simulink library "Contact_Forces_Lib"  (R2024a)
settings: Solver=ode45  StartTime=0.0  StopTime=10.0  RelTol=1e-3  EnableMultiTasking=on
undefined symbols (not defined in the file or in its folder): b_contact, custom_param_1, custom_param_2, Extr_Data_Ring, k_contact, l_cone, length_cylinder, length_tube, mu_kinetic, mu_static, pen_exponent, pen_full_damp_F, rad_s_cone, radius_cylinder, radius_tube, v_thr, X, Y, Z
libraries: nesl_utility x197, sm_lib x115, $bdroot x72, simulink x20, fl_lib x4
(part 4 of 12)

== system Contact_Forces_Lib/3D/Composite Forces ==
  Face to Belt Faces Force : Subsystem  mask(Face to Belt Faces Force){PlaB_x=4, PlaB_y=1, PlaB_z=0.1, FacF_x=0.6, FacF_y=0.6, FacF_z=-0.6/2, FacF_rSph=0.03, force_law_pla2pla=Linear, k_contact_pla2pla=1e4, b_contact_pla2pla=1e2, pen_full_damp_F_pla2pla=1e-4, pen_exponent_pla2pla=1, friction_law_pla2pla=Stick-Slip Continuous, mu_kinetic_pla2pla=0.5, mu_static_pla2pla=0.7, v_thr_pla2pla=0.001, vis_on_pla2pla=off, vis_opc_en_box2box=0, vis_len_plaLz=0.0005, vis_clr=[0.9 0.2 0.2], vis_opc=0.7}
      mask prompts: PlaB_x "PlaB Length x (m)"; PlaB_y "PlaB Length y (m)"; PlaB_z "PlaB Depth to Reference Frame (m)"; FacF_x "FacF Length x (m)"; FacF_y "FacF Length y (m)"; FacF_z "FacF Depth to Reference Frame (m) (+/-)"; FacF_rSph "FacF Sphere Radius"; force_law_pla2pla "Force Law"; k_contact_pla2pla "Contact Stiffness (N/m)"; b_contact_pla2pla "Contact Damping (N/(m/s))"; pen_full_damp_F_pla2pla "Penetration for full damping (m)"; pen_exponent_pla2pla "Penetration exponent (>=1)"; friction_law_pla2pla "Friction Law"; mu_kinetic_pla2pla "Coefficient of Kinetic Friction"; mu_static_pla2pla "Coefficient of Static Friction"; v_thr_pla2pla "Velocity Threshold (m/s)"; vis_on_pla2pla "Visualize Contact Surfaces"; vis_opc_en_box2box "Visualize Opacity Enable"; vis_len_plaLz "Depth Plane Surface Element (Z-Axis) (m)"; vis_clr "Color of Surface Element (RGB)"; vis_opc "Opacity of Surface Element (0-1)"
      mask help:
      | This subsystem models planar contact forces between a square face and a conveyor belt.  The conveyor belt moves at the speed specified by the input signal in m/s.  Velocity can be specified along x or y and affects upper and lower surfaces of the belt.
      |
      | Frame connected to PlaB port:
      | 1. Located at midpoint of plane (x, y, and z).
      | 2. Z-axis is normal to the surfaces where force is active.
      |
      | Frame connected to the FacF port:
      | 1. Located at midpoint of box (x, y, and z).
      | 2. Z-axis is normal to the surfaces where force is active.
      |
      | Output signal is a bus with intermediate calculations and total force.
      mask init:
      | f=Simulink.FindOptions('FollowLinks',0,'LookUnderMasks','none','RegExp',1);
      | CR_bpth=Simulink.findBlocks(gcb,'friction_law','.*',f);
      | if(~isempty(CR_bpth))
      |     temp_frlaw = get_param(gcb,'friction_law_pla2pla');
      |     for i=1:length(CR_bpth)
      |         set_param(CR_bpth(i),'friction_law',temp_frlaw);
      |     end
      |     clear temp_frlaw
      | 
      |     temp_forcelaw = get_param(gcb,'force_law_pla2pla');
      |     for i=1:length(CR_bpth)
      |         set_param(CR_bpth(i),'force_law',temp_forcelaw);
      |     end
      |     clear temp_forcelaw
      | 
      |     temp_vis_on = get_param(gcb,'vis_on_pla2pla');
      |     for i=1:length(CR_bpth)
      |         set_param(CR_bpth(i),'vis_on',temp_vis_on);
      |     end
      |     clear temp_vis_on
      | end
      mask Help: web(which('Face_to_Plane_Contact.html'));
      mask TypeOptions force_law_pla2pla: Linear | Nonlinear
      mask Callback force_law_pla2pla:
      | maskObj = Simulink.Mask.get(gcb);
      | pfd_h = maskObj.getParameter('pen_full_damp_F_pla2pla');
      | pex_h = maskObj.getParameter('pen_exponent_pla2pla');
      | if strcmp(get_param(gcb,'force_law_pla2pla'),'Linear')
      |     pfd_h.Visible = 'off';
      |     pex_h.Visible = 'off';
      | elseif strcmp(get_param(gcb,'force_law_pla2pla'),'Nonlinear')
      |     pfd_h.Visible = 'on';
      |     pex_h.Visible = 'on';
      | end
      mask TypeOptions friction_law_pla2pla: None | Stick-Slip Continuous
      mask Callback friction_law_pla2pla:
      | maskObj = Simulink.Mask.get(gcb);
      | muk_h = maskObj.getParameter('mu_kinetic_pla2pla');
      | mus_h = maskObj.getParameter('mu_static_pla2pla');
      | vth_h = maskObj.getParameter('v_thr_pla2pla');
      | if strcmp(get_param(gcb,'friction_law_pla2pla'),'None')
      |     muk_h.Visible = 'off';
      |     mus_h.Visible = 'off';
      |     vth_h.Visible = 'off';
      | elseif strcmp(get_param(gcb,'friction_law_pla2pla'),'Stick-Slip Continuous')
      |     muk_h.Visible = 'on';
      |     mus_h.Visible = 'on';
      |     vth_h.Visible = 'on';
      | end
      | clear maskObj
      mask Callback vis_on_pla2pla:
      | maskObj = Simulink.Mask.get(gcb);
      | vis_clr_h = maskObj.getParameter('vis_clr');
      | vis_opc_h = maskObj.getParameter('vis_opc');
      | vis_len_plaLz_h = maskObj.getParameter('vis_len_plaLz');
      | if strcmp(get_param(gcb,'vis_on_pla2pla'),'off')
      |     vis_len_plaLz_h.Visible = 'off';
      |     vis_clr_h.Visible = 'off';
      |     vis_opc_h.Visible = 'off';
      | elseif strcmp(get_param(gcb,'vis_on_pla2pla'),'on')
      |     vis_len_plaLz_h.Visible = 'on';
      |     vis_clr_h.Visible = 'on';
      |     vis_opc_h.Visible = 'on';
      | end
      | clear maskObj vis_clr_h vis_opc_h
      | clear vis_len_plaLz_h
      mask DialogControl Container6 Prompt: Dimensions
      mask DialogControl Container7 Prompt: Contact
      mask DialogControl Container9 Prompt: Friction
      mask DialogControl Vis_Cont Prompt: Visual
      mask Display: image('Face_to_Belt_Faces_IMAGE.jpg');
  Face to Plane Force : Subsystem  mask(Face to Plane Force){PlaB_x=1, PlaB_y=1, PlaB_z=0.05, FacF_x=0.1, FacF_y=0.1, FacF_z=0.05, FacF_rSph=0.01, force_law_pla2pla=Linear, k_contact_pla2pla=1e4, b_contact_pla2pla=1e2, pen_full_damp_F_pla2pla=1e-4, pen_exponent_pla2pla=1, friction_law_pla2pla=None, mu_kinetic_pla2pla=0.5, mu_static_pla2pla=0.7, v_thr_pla2pla=0.001, vis_on_pla2pla=off, vis_opc_en_box2box=0, vis_len_plaLz=0.005, vis_clr=[0.9 0.2 0.2], vis_opc=0.7}
      mask prompts: PlaB_x "PlaB Length x (m)"; PlaB_y "PlaB Length y (m)"; PlaB_z "PlaB Depth to Reference Frame (m)"; FacF_x "FacF Length x (m)"; FacF_y "FacF Length y (m)"; FacF_z "FacF Depth to Reference Frame (m) (+/-)"; FacF_rSph "FacF Sphere Radius"; force_law_pla2pla "Force Law"; k_contact_pla2pla "Contact Stiffness (N/m)"; b_contact_pla2pla "Contact Damping (N/(m/s))"; pen_full_damp_F_pla2pla "Penetration for full damping (m)"; pen_exponent_pla2pla "Penetration exponent (>=1)"; friction_law_pla2pla "Friction Law"; mu_kinetic_pla2pla "Coefficient of Kinetic Friction"; mu_static_pla2pla "Coefficient of Static Friction"; v_thr_pla2pla "Velocity Threshold (m/s)"; vis_on_pla2pla "Visualize Contact Surfaces"; vis_opc_en_box2box "Visualize Opacity Enable"; vis_len_plaLz "Depth Plane Surface Element (Z-Axis) (m)"; vis_clr "Color of Surface Element (RGB)"; vis_opc "Opacity of Surface Element (0-1)"
      mask help:
      | This subsystem implements a contact force between a plane and a square face. The plane is assumed significantly larger than the face such that the edges will never intersect.  The force is active above and below the plane and face.
      |
      | Frame connected to PlaB port:
      | 1. Located at midpoint of plane (x, y, and z).
      | 2. Z-axis is normal to the surfaces where force is active.
      |
      | Frame connected to the FacF port:
      | 1. Located at midpoint of box (x, y, and z).
      | 2. Z-axis is normal to the surfaces where force is active.
      |
      | Output signal is a bus with intermediate calculations and total force.
      mask init:
      | f=Simulink.FindOptions('FollowLinks',0,'LookUnderMasks','none','RegExp',1);
      | CR_bpth=Simulink.findBlocks(gcb,'friction_law','.*',f);
      | 
      | if(~isempty(CR_bpth))
      |     temp_frlaw = get_param(gcb,'friction_law_pla2pla');
      |     for i=1:length(CR_bpth)
      |         set_param(CR_bpth(i),'friction_law',temp_frlaw);
      |     end
      |     clear temp_frlaw
      | 
      |     temp_forcelaw = get_param(gcb,'force_law_pla2pla');
      |     for i=1:length(CR_bpth)
      |         set_param(CR_bpth(i),'force_law',temp_forcelaw);
      |     end
      |     clear temp_forcelaw
      | 
      |     temp_vis_on = get_param(gcb,'vis_on_pla2pla');
      |     for i=1:length(CR_bpth)
      |         set_param(CR_bpth(i),'vis_on',temp_vis_on);
      |     end
      |     clear temp_vis_on
      | end
      mask Help: web(which('Face_to_Plane_Contact.html'));
      mask TypeOptions force_law_pla2pla: Linear | Nonlinear
      mask Callback force_law_pla2pla:
      | maskObj = Simulink.Mask.get(gcb);
      | pfd_h = maskObj.getParameter('pen_full_damp_F_pla2pla');
      | pex_h = maskObj.getParameter('pen_exponent_pla2pla');
      | if strcmp(get_param(gcb,'force_law_pla2pla'),'Linear')
      |     pfd_h.Visible = 'off';
      |     pex_h.Visible = 'off';
      | elseif strcmp(get_param(gcb,'force_law_pla2pla'),'Nonlinear')
      |     pfd_h.Visible = 'on';
      |     pex_h.Visible = 'on';
      | end
      mask TypeOptions friction_law_pla2pla: None | Stick-Slip Continuous
      mask Callback friction_law_pla2pla:
      | maskObj = Simulink.Mask.get(gcb);
      | muk_h = maskObj.getParameter('mu_kinetic_pla2pla');
      | mus_h = maskObj.getParameter('mu_static_pla2pla');
      | vth_h = maskObj.getParameter('v_thr_pla2pla');
      | if strcmp(get_param(gcb,'friction_law_pla2pla'),'None')
      |     muk_h.Visible = 'off';
      |     mus_h.Visible = 'off';
      |     vth_h.Visible = 'off';
      | elseif strcmp(get_param(gcb,'friction_law_pla2pla'),'Stick-Slip Continuous')
      |     muk_h.Visible = 'on';
      |     mus_h.Visible = 'on';
      |     vth_h.Visible = 'on';
      | end
      | clear maskObj
      mask Callback vis_on_pla2pla:
      | maskObj = Simulink.Mask.get(gcb);
      | vis_clr_h = maskObj.getParameter('vis_clr');
      | vis_opc_h = maskObj.getParameter('vis_opc');
      | vis_len_plaLz_h = maskObj.getParameter('vis_len_plaLz');
      | if strcmp(get_param(gcb,'vis_on_pla2pla'),'off')
      |     vis_len_plaLz_h.Visible = 'off';
      |     vis_clr_h.Visible = 'off';
      |     vis_opc_h.Visible = 'off';
      | elseif strcmp(get_param(gcb,'vis_on_pla2pla'),'on')
      |     vis_len_plaLz_h.Visible = 'on';
      |     vis_clr_h.Visible = 'on';
      |     vis_opc_h.Visible = 'on';
      | end
      | clear maskObj vis_clr_h vis_opc_h
      | clear vis_len_plaLz_h
      mask DialogControl Container6 Prompt: Dimensions
      mask DialogControl Container7 Prompt: Contact
      mask DialogControl Container9 Prompt: Friction
      mask DialogControl Vis_Cont Prompt: Visual
      mask Display: image('Face_to_Plane_Contact_IMAGE.jpg');
  Sphere to Belt Force : Subsystem  mask(Sphere to Belt Force){sph_rad=1.6, belt_h=1, belt_w=3, belt_l=10, force_law_sph2bel=Linear, k_contact_sph2bel=5e5, b_contact_sph2bel=1e6, pen_full_damp_F_sph2bel=1*1e-2, pen_exponent_sph2bel=1, friction_law_sph2bel=Stick-Slip Continuous, mu_kinetic_sph2bel=0.5, mu_static_sph2bel=0.7, v_thr_sph2bel=1e-3, vis_on_sph2bel=off, vis_opc_en_sph2bel=0, vis_depth_sph2bel=1*0.01, vis_clr=[0.9 0.2 0.2], vis_opc=0.7}
      mask prompts: sph_rad "Sphere Radius (m)"; belt_h "Belt Height (m)"; belt_w "Belt Width (m)"; belt_l "Belt Length (m)"; force_law_sph2bel "Force Law"; k_contact_sph2bel "Contact Stiffness (N/m)"; b_contact_sph2bel "Contact Damping (N/(m/s))"; pen_full_damp_F_sph2bel "Penetration for full damping (m)"; pen_exponent_sph2bel "Penetration exponent (>=1)"; friction_law_sph2bel "Friction Law"; mu_kinetic_sph2bel "Coefficient of Kinetic Friction"; mu_static_sph2bel "Coefficient of Static Friction"; v_thr_sph2bel "Velocity Threshold (m/s)"; vis_on_sph2bel "Visualize Contact Surfaces"; vis_opc_en_sph2bel "Visualize Opacity Enable"; vis_depth_sph2bel "Depth Surface Element (m)"; vis_clr "Color of Surface Element (RGB)"; vis_opc "Opacity of Surface Element (0-1)"
      mask help:
      | This subsystem models contact forces between a sphere and a conveyor belt.  The conveyor belt moves at the speed specified by the input signal in m/s.  The speed and affects upper and lower surfaces of the belt as well as the ends.
      |
      | Frame connected to BelB port:
      | 1. Located at midpoint of plane (x, y, and z).
      | 2. Z-axis is normal to the surfaces where force is active.
      |
      | Frame connected to the SphF port:
      | 1. Located at center of sphere.
      | 2. Orientation does not matter.
      |
      | Output signal is a bus with intermediate calculations and total force. Click Help for a diagram describing this force.
      mask init:
      | f=Simulink.FindOptions('FollowLinks',0,'LookUnderMasks','none','RegExp',1);
      | CR_bpth=Simulink.findBlocks(gcb,'friction_law','.*',f);
      | 
      | if(~isempty(CR_bpth))
      |     temp_frlaw = get_param(gcb,'friction_law_sph2bel');
      |     for i=1:length(CR_bpth)
      |         set_param(CR_bpth(i),'friction_law',temp_frlaw);
      |     end
      |     clear temp_frlaw
      | 
      |     temp_forcelaw = get_param(gcb,'force_law_sph2bel');
      |     for i=1:length(CR_bpth)
      |         set_param(CR_bpth(i),'force_law',temp_forcelaw);
      |     end
      |     clear temp_forcelaw
      | 
      |     temp_vis_on = get_param(gcb,'vis_on_sph2bel');
      |     for i=1:length(CR_bpth)
      |         set_param(CR_bpth(i),'vis_on',temp_vis_on);
      |     end
      |     clear temp_vis_on
      | end
      mask Help: web(which('Sphere_to_Belt_Contact.html'));
      mask TypeOptions force_law_sph2bel: Linear | Nonlinear
      mask Callback force_law_sph2bel:
      | maskObj = Simulink.Mask.get(gcb);
      | pfd_h = maskObj.getParameter('pen_full_damp_F_sph2bel');
      | pex_h = maskObj.getParameter('pen_exponent_sph2bel');
      | if strcmp(get_param(gcb,'force_law_sph2bel'),'Linear')
      |     pfd_h.Visible = 'off';
      |     pex_h.Visible = 'off';
      | elseif strcmp(get_param(gcb,'force_law_sph2bel'),'Nonlinear')
      |     pfd_h.Visible = 'on';
      |     pex_h.Visible = 'on';
      | end
      mask Callback pen_full_damp_F_sph2bel:
      | maskObj = Simulink.Mask.get(gcb);
      | pfd_h = maskObj.getParameter('pen_full_damp_F_sph2bel');
      | pex_h = maskObj.getParameter('pen_exponent_sph2bel');
      | if strcmp(get_param(gcb,'force_law_sph2bel'),'Linear')
      |     pfd_h.Visible = 'off';
      |     pex_h.Visible = 'off';
      | elseif strcmp(get_param(gcb,'force_law_sph2bel'),'Nonlinear')
      |     pfd_h.Visible = 'on';
      |     pex_h.Visible = 'on';
      | end
      mask TypeOptions friction_law_sph2bel: None | Stick-Slip Continuous
      mask Callback friction_law_sph2bel:
      | maskObj = Simulink.Mask.get(gcb);
      | muk_h = maskObj.getParameter('mu_kinetic_sph2bel');
      | mus_h = maskObj.getParameter('mu_static_sph2bel');
      | vth_h = maskObj.getParameter('v_thr_sph2bel');
      | if strcmp(get_param(gcb,'friction_law_sph2bel'),'None')
      |     muk_h.Visible = 'off';
      |     mus_h.Visible = 'off';
      |     vth_h.Visible = 'off';
      | elseif strcmp(get_param(gcb,'friction_law_sph2bel'),'Stick-Slip Continuous')
      |     muk_h.Visible = 'on';
      |     mus_h.Visible = 'on';
      |     vth_h.Visible = 'on';
      | end
      | clear maskObj
      mask Callback vis_on_sph2bel:
      | maskObj = Simulink.Mask.get(gcb);
      | vis_clr_h = maskObj.getParameter('vis_clr');
      | vis_opc_h = maskObj.getParameter('vis_opc');
      | vis_depth_sph2bel_h = maskObj.getParameter('vis_depth_sph2bel');
      | if strcmp(get_param(gcb,'vis_on_sph2bel'),'off')
      |     vis_depth_sph2bel_h.Visible = 'off';
      |     vis_clr_h.Visible = 'off';
      |     vis_opc_h.Visible = 'off';
      | elseif strcmp(get_param(gcb,'vis_on_sph2bel'),'on')
      |     vis_depth_sph2bel_h.Visible = 'on';
      |     vis_clr_h.Visible = 'on';
      |     vis_opc_h.Visible = 'on';
      | end
      | clear maskObj vis_clr_h vis_opc_h
      | clear vis_depth_sph2bel_h
      mask DialogControl cont_dimensions Prompt: Dimensions
      mask DialogControl cont_contact Prompt: Contact
      mask DialogControl cont_friction Prompt: Friction
      mask DialogControl cont_vis Prompt: Visual
      mask Display: image('Sphere_to_Belt_IMAGE.jpg');

== system Contact_Forces_Lib/3D/Prototype ==
  note: These blocks are prototypes, and will change in future releases.
      | They are provided as an example.
  Cone in Ring Force : Subsystem  mask{r_cyl=radius_cylinder, l_cyl=length_cylinder, r_tube=radius_tube, l_tube=length_tube, rl=radius_cylinder, rs=rad_s_cone, lc=l_cone, k_stiff=k_contact, b_damp=b_contact, n=500}
      mask prompts: r_cyl "Cylinder radius (m)"; l_cyl "Cylinder length"; r_tube "Tube radius (m)"; l_tube "Tube length (m)"; rl "Cone Large radius (m)"; rs "Cone Small radius (m)"; lc "Cone Length"; k_stiff "Spring Stifness (N/m)"; b_damp "Damping (Ns/m)"; n "Number of discrete points"
      mask DialogControl Dim Prompt: Dimensions
      mask DialogControl contact Prompt: Contact Forces
      mask Display:
      | port_label('LConn',1,'TubB');
      | port_label('RConn',1,'CylF');
  Cylinder In Ring Force : Subsystem  mask{r_cyl=radius_cylinder, l_cyl=length_cylinder, r_tube=radius_tube, l_tube=length_tube, k_stiff=k_contact, b_damp=b_contact, n=500, mu_kinetic=mu_kinetic, mu_static=mu_static, v_thr=v_thr}
      mask prompts: r_cyl "Cylinder radius (m)"; l_cyl "Cylinder length"; r_tube "Tube radius (m)"; l_tube "Tube length (m)"; k_stiff "Spring Stifness (N/m)"; b_damp "Damping (Ns/m)"; n "Number of discrete points"; mu_kinetic "Coefficient of Kinetic Friction"; mu_static "Coefficient of Static Friction"; v_thr "Velocity Threshold (m/s)"
      mask DialogControl Dim Prompt: Dimensions
      mask DialogControl contact Prompt: Contact Forces
      mask DialogControl Fric Prompt: Friction
      mask Display:
      | port_label('LConn',1,'TubB');
      | port_label('RConn',1,'CylF');
      | port_label('output',1,'Out');

== system Contact_Forces_Lib/3D/Sphere in Sphere Force ==
  Bus Creator : BusCreator  Inputs=2
  Bus Creator1 : BusCreator  Inputs=7
  Calculate Penetration : Subsystem
  External Force and Torque SphB : sm_lib/Forces and Torques/External Force and Torque  EnableForceX=off  EnableForceY=off  EnableForceZ=off  EnableForce=on  ForceResolutionFrame=AttachedFrame  EnableTorqueX=off  EnableTorqueY=off  EnableTorqueZ=off  EnableTorque=on  TorqueResolutionFrame=AttachedFrame
  External Force and Torque SphF : sm_lib/Forces and Torques/External Force and Torque  EnableForceX=off  EnableForceY=off  EnableForceZ=off  EnableForce=on  ForceResolutionFrame=AttachedFrame  EnableTorqueX=off  EnableTorqueY=off  EnableTorqueZ=off  EnableTorque=on  TorqueResolutionFrame=AttachedFrame
  Ff : Subsystem
  Fn : Subsystem
  Force Law : $bdroot/Force Law  SystemSampleTime=-1  LabelModeActiveChoice=Linear  VariantActivationTime=update diagram  AllowFlexibleInterface=on  Latency=0  AutoFrameSizeCalculation=off
  Gain1 : Gain  Gain=-1
  Sensing : Subsystem
  Simulink-PS Converter{1..4} (4 alike) : nesl_utility/Simulink-PS Converter  PhysicalDomain=network_engine_domain  SubClassName=ps_input  LeftPortType=input  RightPortType=output  PseudoPeriodic=off  Frequencies=[]  NoiseDistribution=none  NoiseParameters=[]  Unit=1  AffineConversion=off  FilteringAndDerivatives=zero  SimscapeFilterOrder=1  InputFilterTimeConstant=0.005  UdotUserProvided=1
  Sum : Sum
  Sum2 : Sum
  Visual SphB : sm_lib/Body Elements/Spherical Solid  SphereRadius=max(sphB_rad,1e-8)  SphereRadiusUnits=m  ExportEntireGeometry=off  InertiaType=CalculateFromGeometry  BasedOnType=Density  Density=0  DensityUnits=kg/(m^3)  Mass=1  MassUnits=kg  CenterOfMass=[0 0 0]  CenterOfMassUnits=m  MomentsOfInertia=[1 1 1]  MomentsOfInertiaUnits=kg*m^2  ProductsOfInertia=[0 0 0]  ProductsOfInertiaUnits=kg*m^2  GraphicType=FromGeometry  MarkerShape=Sphere  MarkerSize=10  GraphicVisPropType=SimpleVisualProperties  GraphicDiffuseColor=vis_clr  GraphicOpacity=vis_opc*vis_opc_en  GraphicSpecularColor=[0.5 0.5 0.5 1.0]  GraphicAmbientColor=[0.15 0.15 0.15 1.0]  GraphicEmissiveColor=[0.0 0.0 0.0 1.0]  GraphicShininess=75  DoExposeReferenceFrame=on  SerializedFrames=<Frames/>
  Visual SphF : sm_lib/Body Elements/Spherical Solid  SphereRadius=max(sphF_rad,1e-8)  SphereRadiusUnits=m  ExportEntireGeometry=off  InertiaType=CalculateFromGeometry  BasedOnType=Density  Density=0  DensityUnits=kg/(m^3)  Mass=1  MassUnits=kg  CenterOfMass=[0 0 0]  CenterOfMassUnits=m  MomentsOfInertia=[1 1 1]  MomentsOfInertiaUnits=kg*m^2  ProductsOfInertia=[0 0 0]  ProductsOfInertiaUnits=kg*m^2  GraphicType=FromGeometry  MarkerShape=Sphere  MarkerSize=10  GraphicVisPropType=SimpleVisualProperties  GraphicDiffuseColor=vis_clr  GraphicOpacity=vis_opc*vis_opc_en  GraphicSpecularColor=[0.5 0.5 0.5 1.0]  GraphicAmbientColor=[0.15 0.15 0.15 1.0]  GraphicEmissiveColor=[0.0 0.0 0.0 1.0]  GraphicShininess=75  DoExposeReferenceFrame=on  SerializedFrames=<Frames/>
  SphF : PMIOPort  Side=Left
  SphB : PMIOPort  Port=2  Side=Right
  Out : Outport  VectorParamsAs1DForOutWhenUnconnected=off
  wires:
  Ff/5(Ff) -> Bus Creator1/7  "Friction Force"
  Bus Creator1/1 -> Out/1
  Bus Creator/1 -> Bus Creator1/1  "Frame Sep"
  Ff/3(FSphB) -> Sum2/2
  Fn/2(FSphF) -> Sum/1
  Sensing/4(dvect) -> Fn/4(dvect), Ff/3(dvect)
  Sensing/6(w) -> Ff/5(w)
  Sensing/5(v) -> Ff/4(v)
  Ff/1(FSphF) -> Sum/2
  Force Law/2 -> Fn/3(DamF), Gain1/1
  Sensing/1(R) -> Ff/2(R), Fn/1(R)
  Force Law/1 -> Fn/2(SprF), Bus Creator1/5  "Spr Force"
  Fn/3(FSphB) -> Sum2/1, Ff/1(Fn)  "Normal Force"
  Calculate Penetration/2(Pen Vel) -> Force Law/2, Bus Creator1/3  "Penetration Vel"
  Calculate Penetration/1(Pen) -> Force Law/1, Bus Creator1/2  "Penetration"
  Sum/1 -> Simulink-PS Converter2/1
  Sum2/1 -> Simulink-PS Converter3/1
  Sensing/2(dst) -> Calculate Penetration/1(dst), Bus Creator/1  "dst"
  Sensing/3(vdst) -> Calculate Penetration/2(vdst), Bus Creator/2  "vdst"
  Ff/2(TSphF) -> Simulink-PS Converter1/1
  Ff/4(TSphB) -> Simulink-PS Converter4/1
  Fn/1(Fn) -> Bus Creator1/6  "Normal Force"
  Gain1/1 -> Bus Creator1/4  "Damp Force"
  connections:
  Sensing/LConn1 -- Visual SphF/RConn1 -- External Force and Torque SphF/RConn1 -- SphF/RConn1
  SphB/RConn1 -- External Force and Torque SphB/RConn1 -- Visual SphB/RConn1 -- Sensing/LConn2
  Simulink-PS Converter2/RConn1 -- External Force and Torque SphF/LConn1
  Simulink-PS Converter1/RConn1 -- External Force and Torque SphF/LConn2
  Simulink-PS Converter3/RConn1 -- External Force and Torque SphB/LConn1
  Simulink-PS Converter4/RConn1 -- External Force and Torque SphB/LConn2

== system Contact_Forces_Lib/3D/Sphere to Cone Force ==
  Bus Creator1 : BusCreator  Inputs=3
  Check Active : Subsystem
  Demux : Subsystem
  External Force and Torque SphF : sm_lib/Forces and Torques/External Force and Torque  EnableForceX=on  EnableForceY=on  EnableForceZ=on  EnableForce=off  ForceResolutionFrame=AttachedFrame  EnableTorqueX=off  EnableTorqueY=off  EnableTorqueZ=off  EnableTorque=on  TorqueResolutionFrame=AttachedFrame
  External Force and Torque TubB : sm_lib/Forces and Torques/External Force and Torque  EnableForceX=on  EnableForceY=on  EnableForceZ=on  EnableForce=off  ForceResolutionFrame=AttachedFrame  EnableTorqueX=off  EnableTorqueY=off  EnableTorqueZ=off  EnableTorque=on  TorqueResolutionFrame=AttachedFrame
  Forces : Subsystem
  If1 : If
  Merge : Merge  InitialOutput=0  InputPortOffsets=0
  No Force : Subsystem
  Sensing : Subsystem
  Set Output : Subsystem
  Transform Active Angle : sm_lib/Frames and Transforms/Rigid Transform  RotationMethod=StandardAxis  FollAlignAxisA=+X  BaseAlignAxisA=+Y  FollAlignAxisB=+Y  BaseAlignAxisB=+Z  RotationStandardAxis=+Z  RotationAngle=(active_angle(2)+active_angle(1))/2  RotationAngleUnits=deg  RotationArbitraryAxis=[0 0 1]  RotationSequenceAxes=FollowerAxes  RotationSequence=XYX  RotationSequenceAngles=[0 0 0]  RotationSequenceAnglesUnits=deg  RotationMatrix=[1 0 0; 0 1 0; 0 0 1]  Quaternion=[1 0 0 0]  TranslationMethod=None  TranslationCartesianOffset=[0 0 0]  TranslationCartesianOffsetUnits=m  TranslationStandardAxis=+Z  TranslationStandardOffset=0  TranslationStandardOffsetUnits=m  TranslationROffset=0  TranslationROffsetUnits=m  TranslationThetaOffset=0  TranslationThetaOffsetUnits=deg  TranslationZOffset=0  TranslationZOffsetUnits=m
  Visual ConB Inner : sm_lib/Body Elements/Revolved Solid  RevolutionCrossSection=frcon_xsec_in  RevolutionCrossSectionUnits=m  RevolutionExtent=Custom  RevolutionAngle=active_angle(2)-active_angle(1)  RevolutionAngleUnits=deg  ExportConvexHullGeometry=off  InertiaType=CalculateFromGeometry  BasedOnType=Density  Density=0  DensityUnits=kg/(m^3)  Mass=1  MassUnits=kg  CenterOfMass=[0 0 0]  CenterOfMassUnits=m  MomentsOfInertia=[1 1 1]  MomentsOfInertiaUnits=kg*m^2  ProductsOfInertia=[0 0 0]  ProductsOfInertiaUnits=kg*m^2  GraphicType=FromGeometry  MarkerShape=Sphere  MarkerSize=10  GraphicVisPropType=SimpleVisualProperties  GraphicDiffuseColor=vis_clr  GraphicOpacity=vis_opc*vis_opc_en  GraphicSpecularColor=[0.5 0.5 0.5 1.0]  GraphicAmbientColor=[0.15 0.15 0.15 1.0]  GraphicEmissiveColor=[0.0 0.0 0.0 1.0]  GraphicShininess=75  DoExposeReferenceFrame=on  SerializedFrames=<Frames/>
  Visual ConB Outer : sm_lib/Body Elements/Revolved Solid  RevolutionCrossSection=frcon_xsec_out  RevolutionCrossSectionUnits=m  RevolutionExtent=Custom  RevolutionAngle=active_angle(2)-active_angle(1)  RevolutionAngleUnits=deg  ExportConvexHullGeometry=off  InertiaType=CalculateFromGeometry  BasedOnType=Density  Density=0  DensityUnits=kg/(m^3)  Mass=1  MassUnits=kg  CenterOfMass=[0 0 0]  CenterOfMassUnits=m  MomentsOfInertia=[1 1 1]  MomentsOfInertiaUnits=kg*m^2  ProductsOfInertia=[0 0 0]  ProductsOfInertiaUnits=kg*m^2  GraphicType=FromGeometry  MarkerShape=Sphere  MarkerSize=10  GraphicVisPropType=SimpleVisualProperties  GraphicDiffuseColor=vis_clr  GraphicOpacity=vis_opc*vis_opc_en  GraphicSpecularColor=[0.5 0.5 0.5 1.0]  GraphicAmbientColor=[0.15 0.15 0.15 1.0]  GraphicEmissiveColor=[0.0 0.0 0.0 1.0]  GraphicShininess=75  DoExposeReferenceFrame=on  SerializedFrames=<Frames/>
  Visual SphF : sm_lib/Body Elements/Spherical Solid  SphereRadius=radius_sphere  SphereRadiusUnits=m  ExportEntireGeometry=off  InertiaType=CalculateFromGeometry  BasedOnType=Density  Density=0  DensityUnits=kg/(m^3)  Mass=1  MassUnits=kg  CenterOfMass=[0 0 0]  CenterOfMassUnits=m  MomentsOfInertia=[1 1 1]  MomentsOfInertiaUnits=kg*m^2  ProductsOfInertia=[0 0 0]  ProductsOfInertiaUnits=kg*m^2  GraphicType=FromGeometry  MarkerShape=Sphere  MarkerSize=10  GraphicVisPropType=SimpleVisualProperties  GraphicDiffuseColor=vis_clr  GraphicOpacity=vis_opc*vis_opc_en  GraphicSpecularColor=[0.5 0.5 0.5 1.0]  GraphicAmbientColor=[0.15 0.15 0.15 1.0]  GraphicEmissiveColor=[0.0 0.0 0.0 1.0]  GraphicShininess=75  DoExposeReferenceFrame=on  SerializedFrames=<Frames/>
  SphF : PMIOPort  Tag=PMCPort  Side=Left
  ConB : PMIOPort  Tag=PMCPort  Port=2  Side=Right
  Out : Outport  VectorParamsAs1DForOutWhenUnconnected=off
  wires:
  Sensing/12(vazmy) -> Forces/12(vazmy)
  Sensing/11(vazmx) -> Forces/11(vazmx)
  Check Active/1(En) -> If1/1, Set Output/2(En)
  Set Output/1(Out) -> Out/1
  Bus Creator1/1 -> Set Output/3(FrameSep)  "Frame Sep"
  Forces/2(Out) -> Set Output/1(Frc)
  Sensing/5(vazm) -> Forces/5(vazm)
  Sensing/2(rad) -> Forces/2(rad), Bus Creator1/1  "rad"
  Sensing/8(R) -> Forces/8(R)
  Forces/1(Frc) -> Merge/2
  No Force/1(F) -> Merge/1
  If1/1 -> Forces/Action
  If1/2 -> No Force/Action
  Sensing/4(azm) -> Bus Creator1/3, Forces/4(azm), Check Active/2(azm)  "azm"
  Sensing/3(vrad) -> Forces/3(vrad), Bus Creator1/2  "vrad"
  Sensing/7(wzf) -> Forces/7(wzf)
  Merge/1 -> Demux/1(Frc)  "Total Force"
  Sensing/1(z) -> Forces/1(z), Check Active/1(z)
  Sensing/6(vzf) -> Forces/6(vzf)
  Sensing/9(wxf) -> Forces/9(wxf)
  Sensing/10(wyf) -> Forces/10(wyf)
  connections:
  Transform Active Angle/RConn1 -- Visual ConB Inner/RConn1 -- Visual ConB Outer/RConn1
  Demux/RConn2 -- External Force and Torque SphF/LConn2
  Demux/RConn1 -- External Force and Torque SphF/LConn1
  Demux/RConn5 -- External Force and Torque TubB/LConn1
  Demux/RConn6 -- External Force and Torque TubB/LConn2
  Transform Active Angle/LConn1 -- External Force and Torque TubB/RConn1 -- ConB/RConn1 -- Sensing/LConn2
  Sensing/LConn1 -- SphF/RConn1 -- Visual SphF/RConn1 -- External Force and Torque SphF/RConn1
  Demux/RConn3 -- External Force and Torque SphF/LConn3
  Demux/RConn7 -- External Force and Torque TubB/LConn3
  Demux/RConn8 -- External Force and Torque TubB/LConn4
  Demux/RConn4 -- External Force and Torque SphF/LConn4

== system Contact_Forces_Lib/3D/Sphere to Plane Force ==
  Bus Creator : BusCreator  Inputs=3
  Check Sphere on Plane : Subsystem
  Demux : Subsystem
  Enable Outputs : Subsystem
  External Force and Torque PlaB : sm_lib/Forces and Torques/External Force and Torque  EnableForceX=off  EnableForceY=off  EnableForceZ=off  EnableForce=on  ForceResolutionFrame=AttachedFrame  EnableTorqueX=off  EnableTorqueY=off  EnableTorqueZ=off  EnableTorque=on  TorqueResolutionFrame=AttachedFrame
  External Force and Torque SphF : sm_lib/Forces and Torques/External Force and Torque  EnableForceX=off  EnableForceY=off  EnableForceZ=off  EnableForce=on  ForceResolutionFrame=AttachedFrame  EnableTorqueX=off  EnableTorqueY=off  EnableTorqueZ=off  EnableTorque=on  TorqueResolutionFrame=AttachedFrame
  Forces : Subsystem
  If1 : If  IfExpression=u1>0
  Merge : Merge
  No Force : Subsystem  TreatAsAtomicUnit=on
  Sensing : Subsystem
  Transform nZ : sm_lib/Frames and Transforms/Rigid Transform  RotationMethod=None  FollAlignAxisA=+X  BaseAlignAxisA=+Y  FollAlignAxisB=+Y  BaseAlignAxisB=+Z  RotationStandardAxis=+Z  RotationAngle=0.0  RotationAngleUnits=deg  RotationArbitraryAxis=[0 0 1]  RotationSequenceAxes=FollowerAxes  RotationSequence=XYX  RotationSequenceAngles=[0 0 0]  RotationSequenceAnglesUnits=deg  RotationMatrix=[1 0 0; 0 1 0; 0 0 1]  Quaternion=[1 0 0 0]  TranslationMethod=StandardAxis  TranslationCartesianOffset=[0 0 0]  TranslationCartesianOffsetUnits=m  TranslationStandardAxis=-Z  TranslationStandardOffset=plane_depth-vis_len_plaBz/2  TranslationStandardOffsetUnits=m  TranslationROffset=0  TranslationROffsetUnits=m  TranslationThetaOffset=0  TranslationThetaOffsetUnits=deg  TranslationZOffset=0  TranslationZOffsetUnits=m
  Transform pZ : sm_lib/Frames and Transforms/Rigid Transform  RotationMethod=None  FollAlignAxisA=+X  BaseAlignAxisA=+Y  FollAlignAxisB=+Y  BaseAlignAxisB=+Z  RotationStandardAxis=+Z  RotationAngle=0.0  RotationAngleUnits=deg  RotationArbitraryAxis=[0 0 1]  RotationSequenceAxes=FollowerAxes  RotationSequence=XYX  RotationSequenceAngles=[0 0 0]  RotationSequenceAnglesUnits=deg  RotationMatrix=[1 0 0; 0 1 0; 0 0 1]  Quaternion=[1 0 0 0]  TranslationMethod=StandardAxis  TranslationCartesianOffset=[0 0 0]  TranslationCartesianOffsetUnits=m  TranslationStandardAxis=+Z  TranslationStandardOffset=plane_depth-vis_len_plaBz/2  TranslationStandardOffsetUnits=m  TranslationROffset=0  TranslationROffsetUnits=m  TranslationThetaOffset=0  TranslationThetaOffsetUnits=deg  TranslationZOffset=0  TranslationZOffsetUnits=m
  Visual PlaBnZ : sm_lib/Body Elements/Brick Solid  BrickDimensions=[plane_lenx plane_leny vis_len_plaBz]  BrickDimensionsUnits=m  ExportEntireGeometry=off  InertiaType=CalculateFromGeometry  BasedOnType=Density  Density=0  DensityUnits=kg/(m^3)  Mass=1  MassUnits=kg  CenterOfMass=[0 0 0]  CenterOfMassUnits=m  MomentsOfInertia=[1 1 1]  MomentsOfInertiaUnits=kg*m^2  ProductsOfInertia=[0 0 0]  ProductsOfInertiaUnits=kg*m^2  GraphicType=FromGeometry  MarkerShape=Sphere  MarkerSize=10  GraphicVisPropType=SimpleVisualProperties  GraphicDiffuseColor=vis_clr  GraphicOpacity=vis_opc*vis_opc_en  GraphicSpecularColor=[0.5 0.5 0.5 1.0]  GraphicAmbientColor=[0.15 0.15 0.15 1.0]  GraphicEmissiveColor=[0.0 0.0 0.0 1.0]  GraphicShininess=75  DoExposeReferenceFrame=on  SerializedFrames=<Frames/>
  Visual PlaBpZ : sm_lib/Body Elements/Brick Solid  BrickDimensions=[plane_lenx plane_leny vis_len_plaBz]  BrickDimensionsUnits=m  ExportEntireGeometry=off  InertiaType=CalculateFromGeometry  BasedOnType=Density  Density=0  DensityUnits=kg/(m^3)  Mass=1  MassUnits=kg  CenterOfMass=[0 0 0]  CenterOfMassUnits=m  MomentsOfInertia=[1 1 1]  MomentsOfInertiaUnits=kg*m^2  ProductsOfInertia=[0 0 0]  ProductsOfInertiaUnits=kg*m^2  GraphicType=FromGeometry  MarkerShape=Sphere  MarkerSize=10  GraphicVisPropType=SimpleVisualProperties  GraphicDiffuseColor=vis_clr  GraphicOpacity=vis_opc*vis_opc_en  GraphicSpecularColor=[0.5 0.5 0.5 1.0]  GraphicAmbientColor=[0.15 0.15 0.15 1.0]  GraphicEmissiveColor=[0.0 0.0 0.0 1.0]  GraphicShininess=75  DoExposeReferenceFrame=on  SerializedFrames=<Frames/>
  Visual SphF : sm_lib/Body Elements/Spherical Solid  SphereRadius=max(sphere_rad,1e-8)  SphereRadiusUnits=m  ExportEntireGeometry=off  InertiaType=CalculateFromGeometry  BasedOnType=Density  Density=0  DensityUnits=kg/(m^3)  Mass=1  MassUnits=kg  CenterOfMass=[0 0 0]  CenterOfMassUnits=m  MomentsOfInertia=[1 1 1]  MomentsOfInertiaUnits=kg*m^2  ProductsOfInertia=[0 0 0]  ProductsOfInertiaUnits=kg*m^2  GraphicType=FromGeometry  MarkerShape=Sphere  MarkerSize=10  GraphicVisPropType=SimpleVisualProperties  GraphicDiffuseColor=vis_clr  GraphicOpacity=vis_opc*vis_opc_en  GraphicSpecularColor=[0.5 0.5 0.5 1.0]  GraphicAmbientColor=[0.15 0.15 0.15 1.0]  GraphicEmissiveColor=[0.0 0.0 0.0 1.0]  GraphicShininess=75  DoExposeReferenceFrame=on  SerializedFrames=<Frames/>
  SphF : PMIOPort  Side=Left
  PlaB : PMIOPort  Port=2  Side=Right
  Out : Outport  VectorParamsAs1DForOutWhenUnconnected=off
  wires:
  No Force/1(Frc) -> Merge/1
  If1/2 -> No Force/Action
  If1/1 -> Forces/Action
  Sensing/2(y) -> Check Sphere on Plane/2(y), Bus Creator/2, Forces/2(y)  "y"
  Sensing/1(x) -> Check Sphere on Plane/1(x), Bus Creator/1, Forces/1(x)  "x"
  Sensing/9(vy) -> Forces/9(vy)
  Sensing/8(vx) -> Forces/8(vx)
  Sensing/7(wy) -> Forces/7(wy)
  Sensing/6(wx) -> Forces/6(wx)
  Sensing/3(z) -> Bus Creator/3, Forces/3(z)  "z"
  Sensing/5(R) -> Forces/5(R)
  Sensing/4(vz) -> Forces/4(vz)
  Forces/1(Frc) -> Merge/2
  Merge/1 -> Demux/1(Frc)  "FSph"
  Forces/2(Out) -> Enable Outputs/1(Frc)
  Bus Creator/1 -> Enable Outputs/3(FrameSep)  "Frame Sep"
  Enable Outputs/1(Out) -> Out/1
  Check Sphere on Plane/1(En) -> Enable Outputs/2(En), If1/1
  connections:
  Demux/RConn4 -- External Force and Torque PlaB/LConn2
  Demux/RConn3 -- External Force and Torque PlaB/LConn1
  Demux/RConn2 -- External Force and Torque SphF/LConn2
  Demux/RConn1 -- External Force and Torque SphF/LConn1
  Transform pZ/LConn1 -- Transform nZ/LConn1 -- External Force and Torque PlaB/RConn1 -- Sensing/LConn2 -- PlaB/RConn1
  External Force and Torque SphF/RConn1 -- Visual SphF/RConn1 -- Sensing/LConn1 -- SphF/RConn1
  Transform nZ/RConn1 -- Visual PlaBnZ/RConn1
  Transform pZ/RConn1 -- Visual PlaBpZ/RConn1

== system Contact_Forces_Lib/3D/Sphere to Plane Force Enabled ==
  In : Inport
  Bus Creator : BusCreator  Inputs=3
  Bus Selector1 : BusSelector  OutputSignals=Enable
  Check Sphere on Plane : Subsystem
  Demux : Subsystem
  Enable Outputs : Subsystem
  External Force and Torque PlaB : sm_lib/Forces and Torques/External Force and Torque  EnableForceX=off  EnableForceY=off  EnableForceZ=off  EnableForce=on  ForceResolutionFrame=AttachedFrame  EnableTorqueX=off  EnableTorqueY=off  EnableTorqueZ=off  EnableTorque=on  TorqueResolutionFrame=AttachedFrame
  External Force and Torque SphF : sm_lib/Forces and Torques/External Force and Torque  EnableForceX=off  EnableForceY=off  EnableForceZ=off  EnableForce=on  ForceResolutionFrame=AttachedFrame  EnableTorqueX=off  EnableTorqueY=off  EnableTorqueZ=off  EnableTorque=on  TorqueResolutionFrame=AttachedFrame
  Forces : Subsystem
  If : If  NumInputs=2  IfExpression=(u1 > 0 & u2>0)
  In1 : InportShadow
  Merge : Merge
  No Force : Subsystem  TreatAsAtomicUnit=on
  Sensing : Subsystem
  Transform nZ : sm_lib/Frames and Transforms/Rigid Transform  RotationMethod=None  FollAlignAxisA=+X  BaseAlignAxisA=+Y  FollAlignAxisB=+Y  BaseAlignAxisB=+Z  RotationStandardAxis=+Z  RotationAngle=0.0  RotationAngleUnits=deg  RotationArbitraryAxis=[0 0 1]  RotationSequenceAxes=FollowerAxes  RotationSequence=XYX  RotationSequenceAngles=[0 0 0]  RotationSequenceAnglesUnits=deg  RotationMatrix=[1 0 0; 0 1 0; 0 0 1]  Quaternion=[1 0 0 0]  TranslationMethod=StandardAxis  TranslationCartesianOffset=[0 0 0]  TranslationCartesianOffsetUnits=m  TranslationStandardAxis=-Z  TranslationStandardOffset=plane_depth-vis_len_plaBz/2  TranslationStandardOffsetUnits=m  TranslationROffset=0  TranslationROffsetUnits=m  TranslationThetaOffset=0  TranslationThetaOffsetUnits=deg  TranslationZOffset=0  TranslationZOffsetUnits=m
  Transform pZ : sm_lib/Frames and Transforms/Rigid Transform  RotationMethod=None  FollAlignAxisA=+X  BaseAlignAxisA=+Y  FollAlignAxisB=+Y  BaseAlignAxisB=+Z  RotationStandardAxis=+Z  RotationAngle=0.0  RotationAngleUnits=deg  RotationArbitraryAxis=[0 0 1]  RotationSequenceAxes=FollowerAxes  RotationSequence=XYX  RotationSequenceAngles=[0 0 0]  RotationSequenceAnglesUnits=deg  RotationMatrix=[1 0 0; 0 1 0; 0 0 1]  Quaternion=[1 0 0 0]  TranslationMethod=StandardAxis  TranslationCartesianOffset=[0 0 0]  TranslationCartesianOffsetUnits=m  TranslationStandardAxis=+Z  TranslationStandardOffset=plane_depth-vis_len_plaBz/2  TranslationStandardOffsetUnits=m  TranslationROffset=0  TranslationROffsetUnits=m  TranslationThetaOffset=0  TranslationThetaOffsetUnits=deg  TranslationZOffset=0  TranslationZOffsetUnits=m
  Visual CirF : sm_lib/Body Elements/Spherical Solid  SphereRadius=sphere_rad  SphereRadiusUnits=m  ExportEntireGeometry=off  InertiaType=CalculateFromGeometry  BasedOnType=Density  Density=0  DensityUnits=kg/(m^3)  Mass=1  MassUnits=kg  CenterOfMass=[0 0 0]  CenterOfMassUnits=m  MomentsOfInertia=[1 1 1]  MomentsOfInertiaUnits=kg*m^2  ProductsOfInertia=[0 0 0]  ProductsOfInertiaUnits=kg*m^2  GraphicType=FromGeometry  MarkerShape=Sphere  MarkerSize=10  GraphicVisPropType=SimpleVisualProperties  GraphicDiffuseColor=vis_clr  GraphicOpacity=vis_opc*vis_opc_en  GraphicSpecularColor=[0.5 0.5 0.5 1.0]  GraphicAmbientColor=[0.15 0.15 0.15 1.0]  GraphicEmissiveColor=[0.0 0.0 0.0 1.0]  GraphicShininess=75  DoExposeReferenceFrame=on  SerializedFrames=<Frames/>
  Visual PlaBnZ : sm_lib/Body Elements/Brick Solid  BrickDimensions=[plane_lenx plane_leny vis_len_plaBz]  BrickDimensionsUnits=m  ExportEntireGeometry=off  InertiaType=CalculateFromGeometry  BasedOnType=Density  Density=0  DensityUnits=kg/(m^3)  Mass=1  MassUnits=kg  CenterOfMass=[0 0 0]  CenterOfMassUnits=m  MomentsOfInertia=[1 1 1]  MomentsOfInertiaUnits=kg*m^2  ProductsOfInertia=[0 0 0]  ProductsOfInertiaUnits=kg*m^2  GraphicType=FromGeometry  MarkerShape=Sphere  MarkerSize=10  GraphicVisPropType=SimpleVisualProperties  GraphicDiffuseColor=vis_clr  GraphicOpacity=vis_opc*vis_opc_en  GraphicSpecularColor=[0.5 0.5 0.5 1.0]  GraphicAmbientColor=[0.15 0.15 0.15 1.0]  GraphicEmissiveColor=[0.0 0.0 0.0 1.0]  GraphicShininess=75  DoExposeReferenceFrame=on  SerializedFrames=<Frames/>
  Visual PlaBpZ : sm_lib/Body Elements/Brick Solid  BrickDimensions=[plane_lenx plane_leny vis_len_plaBz]  BrickDimensionsUnits=m  ExportEntireGeometry=off  InertiaType=CalculateFromGeometry  BasedOnType=Density  Density=0  DensityUnits=kg/(m^3)  Mass=1  MassUnits=kg  CenterOfMass=[0 0 0]  CenterOfMassUnits=m  MomentsOfInertia=[1 1 1]  MomentsOfInertiaUnits=kg*m^2  ProductsOfInertia=[0 0 0]  ProductsOfInertiaUnits=kg*m^2  GraphicType=FromGeometry  MarkerShape=Sphere  MarkerSize=10  GraphicVisPropType=SimpleVisualProperties  GraphicDiffuseColor=vis_clr  GraphicOpacity=vis_opc*vis_opc_en  GraphicSpecularColor=[0.5 0.5 0.5 1.0]  GraphicAmbientColor=[0.15 0.15 0.15 1.0]  GraphicEmissiveColor=[0.0 0.0 0.0 1.0]  GraphicShininess=75  DoExposeReferenceFrame=on  SerializedFrames=<Frames/>
  SphF : PMIOPort  Side=Left
  PlaB : PMIOPort  Port=2  Side=Right
  Out : Outport  VectorParamsAs1DForOutWhenUnconnected=off
  wires:
  Check Sphere on Plane/1(En) -> If/2, Enable Outputs/2(En)
  Enable Outputs/1(Out) -> Out/1
  Bus Creator/1 -> Enable Outputs/3(FrameSep)  "Frame Sep"
  Forces/2(Out) -> Enable Outputs/1(Frc)
  Merge/1 -> Demux/1(Frc)  "FSph"
  Forces/1(Frc) -> Merge/2
  Sensing/4(vz) -> Forces/4(vz)
  Sensing/5(R) -> Forces/5(R)
  Sensing/3(z) -> Forces/3(z), Bus Creator/3  "z"
  Sensing/6(wx) -> Forces/6(wx)
  Sensing/7(wy) -> Forces/7(wy)
  Sensing/8(vx) -> Forces/8(vx)
  Sensing/9(vy) -> Forces/9(vy)
  Sensing/1(x) -> Forces/1(x), Bus Creator/1, Check Sphere on Plane/1(x)  "x"
  Sensing/2(y) -> Forces/2(y), Bus Creator/2, Check Sphere on Plane/2(y)  "y"
  If/1 -> Forces/Action
  If/2 -> No Force/Action
  No Force/1(Frc) -> Merge/1
  In/1 -> Bus Selector1/1
  Bus Selector1/1 -> If/1  "<Enable>"
  In1/1 -> Sensing/1(In)
  connections:
  Transform pZ/RConn1 -- Visual PlaBpZ/RConn1
  Transform nZ/RConn1 -- Visual PlaBnZ/RConn1
  SphF/RConn1 -- Sensing/LConn1 -- Visual CirF/RConn1 -- External Force and Torque SphF/RConn1
  PlaB/RConn1 -- Sensing/LConn2 -- External Force and Torque PlaB/RConn1 -- Transform nZ/LConn1 -- Transform pZ/LConn1
  Demux/RConn1 -- External Force and Torque SphF/LConn1
  Demux/RConn2 -- External Force and Torque SphF/LConn2
  Demux/RConn3 -- External Force and Torque PlaB/LConn1
  Demux/RConn4 -- External Force and Torque PlaB/LConn2

== system Contact_Forces_Lib/3D/Sphere to Sphere Force ==
  Bus Creator : BusCreator  Inputs=2
  Bus Creator1 : BusCreator  Inputs=7
  Calculate Penetration : Subsystem
  External Force and Torque SphB : sm_lib/Forces and Torques/External Force and Torque  EnableForceX=off  EnableForceY=off  EnableForceZ=off  EnableForce=on  ForceResolutionFrame=AttachedFrame  EnableTorqueX=off  EnableTorqueY=off  EnableTorqueZ=off  EnableTorque=on  TorqueResolutionFrame=AttachedFrame
  External Force and Torque SphF : sm_lib/Forces and Torques/External Force and Torque  EnableForceX=off  EnableForceY=off  EnableForceZ=off  EnableForce=on  ForceResolutionFrame=AttachedFrame  EnableTorqueX=off  EnableTorqueY=off  EnableTorqueZ=off  EnableTorque=on  TorqueResolutionFrame=AttachedFrame
  Ff : Subsystem
  Fn : Subsystem
  Force Law : $bdroot/Force Law  SystemSampleTime=-1  LabelModeActiveChoice=Linear  VariantActivationTime=update diagram  AllowFlexibleInterface=on  Latency=0  AutoFrameSizeCalculation=off
  Gain1 : Gain  Gain=-1
  Sensing : Subsystem
  Simulink-PS Converter{1..4} (4 alike) : nesl_utility/Simulink-PS Converter  PhysicalDomain=network_engine_domain  SubClassName=ps_input  LeftPortType=input  RightPortType=output  PseudoPeriodic=off  Frequencies=[]  NoiseDistribution=none  NoiseParameters=[]  Unit=1  AffineConversion=off  FilteringAndDerivatives=zero  SimscapeFilterOrder=1  InputFilterTimeConstant=0.005  UdotUserProvided=1
  Sum : Sum
  Sum2 : Sum
  Visual SphB : sm_lib/Body Elements/Spherical Solid  SphereRadius=max(sphB_rad,1e-8)  SphereRadiusUnits=m  ExportEntireGeometry=off  InertiaType=CalculateFromGeometry  BasedOnType=Density  Density=0  DensityUnits=kg/(m^3)  Mass=1  MassUnits=kg  CenterOfMass=[0 0 0]  CenterOfMassUnits=m  MomentsOfInertia=[1 1 1]  MomentsOfInertiaUnits=kg*m^2  ProductsOfInertia=[0 0 0]  ProductsOfInertiaUnits=kg*m^2  GraphicType=FromGeometry  MarkerShape=Sphere  MarkerSize=10  GraphicVisPropType=SimpleVisualProperties  GraphicDiffuseColor=vis_clr  GraphicOpacity=vis_opc*vis_opc_en  GraphicSpecularColor=[0.5 0.5 0.5 1.0]  GraphicAmbientColor=[0.15 0.15 0.15 1.0]  GraphicEmissiveColor=[0.0 0.0 0.0 1.0]  GraphicShininess=75  DoExposeReferenceFrame=on  SerializedFrames=<Frames/>
  Visual SphF : sm_lib/Body Elements/Spherical Solid  SphereRadius=max(sphF_rad,1e-8)  SphereRadiusUnits=m  ExportEntireGeometry=off  InertiaType=CalculateFromGeometry  BasedOnType=Density  Density=0  DensityUnits=kg/(m^3)  Mass=1  MassUnits=kg  CenterOfMass=[0 0 0]  CenterOfMassUnits=m  MomentsOfInertia=[1 1 1]  MomentsOfInertiaUnits=kg*m^2  ProductsOfInertia=[0 0 0]  ProductsOfInertiaUnits=kg*m^2  GraphicType=FromGeometry  MarkerShape=Sphere  MarkerSize=10  GraphicVisPropType=SimpleVisualProperties  GraphicDiffuseColor=vis_clr  GraphicOpacity=vis_opc*vis_opc_en  GraphicSpecularColor=[0.5 0.5 0.5 1.0]  GraphicAmbientColor=[0.15 0.15 0.15 1.0]  GraphicEmissiveColor=[0.0 0.0 0.0 1.0]  GraphicShininess=75  DoExposeReferenceFrame=on  SerializedFrames=<Frames/>
  SphF : PMIOPort  Side=Left
  SphB : PMIOPort  Port=2  Side=Right
  Out : Outport  VectorParamsAs1DForOutWhenUnconnected=off
  wires:
  Fn/1(Fn) -> Bus Creator1/6  "Normal Force"
  Ff/4(TSphB) -> Simulink-PS Converter4/1
  Ff/2(TSphF) -> Simulink-PS Converter1/1
  Sensing/3(vdst) -> Bus Creator/2, Calculate Penetration/2(vdst)  "vdst"
  Sensing/2(dst) -> Bus Creator/1, Calculate Penetration/1(dst)  "dst"
  Sum2/1 -> Simulink-PS Converter3/1
  Sum/1 -> Simulink-PS Converter2/1
  Calculate Penetration/1(Pen) -> Bus Creator1/2, Force Law/1  "Penetration"
  Calculate Penetration/2(Pen Vel) -> Bus Creator1/3, Force Law/2  "Penetration Vel"
  Fn/3(FSphB) -> Sum2/1, Ff/1(Fn)  "Normal Force"
  Force Law/1 -> Bus Creator1/5, Fn/2(SprF)  "Spr Force"
  Sensing/1(R) -> Fn/1(R), Ff/2(R)
  Force Law/2 -> Gain1/1, Fn/3(DamF)
  Ff/1(FSphF) -> Sum/2
  Sensing/5(v) -> Ff/4(v)
  Sensing/6(w) -> Ff/5(w)
  Sensing/4(dvect) -> Fn/4(dvect), Ff/3(dvect)
  Fn/2(FSphF) -> Sum/1
  Ff/3(FSphB) -> Sum2/2
  Bus Creator/1 -> Bus Creator1/1  "Frame Sep"
  Bus Creator1/1 -> Out/1
  Ff/5(Ff) -> Bus Creator1/7  "Friction Force"
  Gain1/1 -> Bus Creator1/4  "Damp Force"
  connections:
  Simulink-PS Converter4/RConn1 -- External Force and Torque SphB/LConn2
  Simulink-PS Converter3/RConn1 -- External Force and Torque SphB/LConn1
  Simulink-PS Converter1/RConn1 -- External Force and Torque SphF/LConn2
  Simulink-PS Converter2/RConn1 -- External Force and Torque SphF/LConn1
  External Force and Torque SphB/RConn1 -- Visual SphB/RConn1 -- SphB/RConn1 -- Sensing/LConn2
  External Force and Torque SphF/RConn1 -- Visual SphF/RConn1 -- Sensing/LConn1 -- SphF/RConn1
